simulink model "SimulationMobileManipulator"  (R2025b)
settings: Solver=FixedStepAuto  StartTime=0.0  StopTime=70  FixedStep=0.01  RelTol=1e-3  EnableMultiTasking=on
libraries: quarc_library x1
settings Model: ExtModeTrigDuration=10000  Creator=prata  LastModifiedBy=prata
settings SolverCC: AlgebraicLoopSolver=TrustRegion  PositivePriorityOrder=on
settings DataIOCC: ReturnWorkspaceOutputs=off
settings OptimizationCC: LifeSpan=inf
settings DebuggingCC: UnconnectedInputMsg=warning  UnconnectedOutputMsg=warning  UnconnectedLineMsg=warning  ArithmeticOperatorsInVariantConditions=warning
settings ModelReferenceCC: EnableRefExpFcnMdlSchedulingChecks=on
settings SFSimCC: SimUseLocalCustomCode=off  CustomCodeUndefinedFunction=UseInterfaceOnly
settings RTWCC: SystemTargetFile=quarc_win64.tlc  TemplateMakefile=quarc_default_tmf  RTWUseLocalCustomCode=off  GPUComputeCapability=3.5  Description=QUARC Win64 Target
settings CodeAppCC: StateflowObjectComments=on
settings STFCustomTargetCC: SystemTargetFile=quarc_win64.tlc  TargetPreCompLibLocation=C:\PROGRA~3\QUARC\lib\2016a\win64\release  TargetLangStandard=C99 (ISO)  DownloadToTarget=on  StopOnOverrun=off  Debug=off
settings GRTTargetCC: ExtMode=on  ExtModeMexFile=quarc_comm  TargetPreCompLibLocation=C:\PROGRA~3\QUARC\lib\2016a\win64\release  ParMdlRefBuildCompliant=off  CompOptLevelCompliant=off  CombineOutputUpdateFcns=off  MatFileLogging=off  CPPClassGenCompliant=off  GRTInterface=on  UseToolchainInfoCompliant=off
settings ConfigComp: CovMetricSettings=dswe

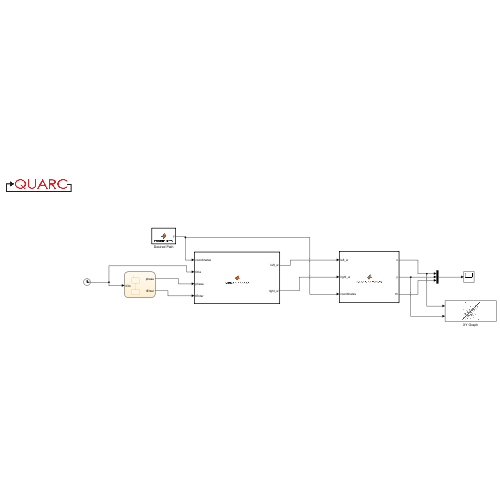
[thumbnail: Simulink's stored preview of the top-level diagram]
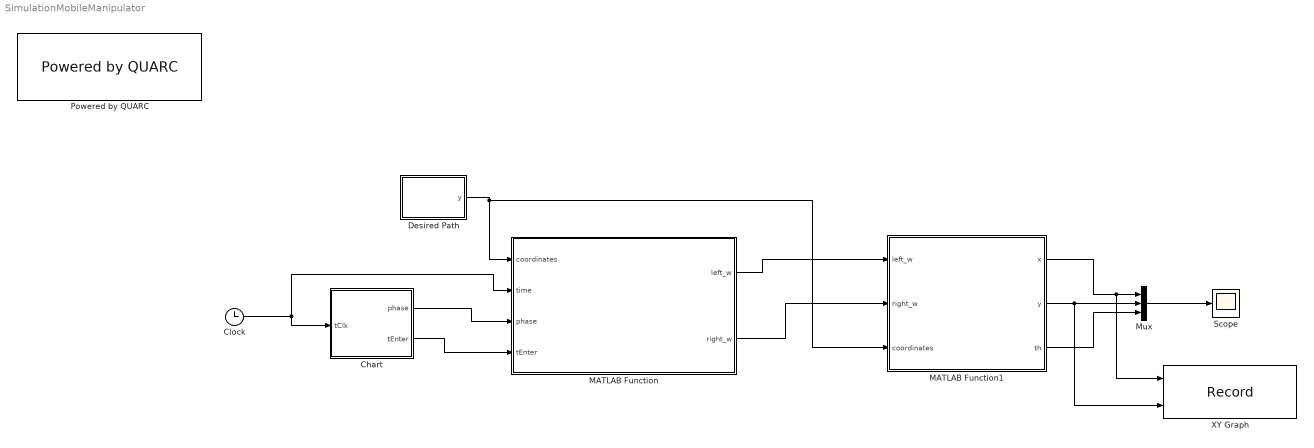
== system SimulationMobileManipulator ==
  Chart : Stateflow chart  TreatAsAtomicUnit=on
  Clock : Clock
  Desired Path : MATLAB Function  TreatAsAtomicUnit=on
  MATLAB Function : MATLAB Function  TreatAsAtomicUnit=on
  MATLAB Function1 : MATLAB Function  TreatAsAtomicUnit=on
  Mux : Mux  Inputs=3
  Powered by QUARC : quarc_library/Logos/Powered by QUARC
  Scope : Scope
      settings: ActiveDisplayYMinimum=-14.807697034096025  ActiveDisplayYMaximum=19.139251197660155
  XY Graph : Record  NumPorts=2.0  FileSettingsInternal="{\"entries\":[{\"content\":{\"excelSettings\":{\"content\":{},\"type\":\"Streamout.ExcelSettings\"},\"parquetSettings\":{\"content\":{},\"type\":\"Streamout.ParquetSettings\"}},\"type\":\"Streamout.FileSettingStorage\",\"uuid\":\"\"}],\"packageUris\":[\"http:\\/\\/schema.mathworks.com\\/mf0\\/streamout_blocks\\/R2020a\"],\"version\":\"1.0\"}"  FrameSettings=[0, 0]  Layout=[1 1]  SignalsInternal="{\"entries\":[{\"content\":{\"signals\":[{\"content\":{\"blockPath\":[],\"dimensions\":[1],\"domain\":\"\",\"lineColor\":\"#a2142f\",\"plots\":[ 1 ],\"port\":1,\"sid\":[\"\"],\"signalID\":1,\"signalName\":\"MATLAB Function1:1\"},\"type\":\"RecordBlkView.Signal\",\"uuid\":\"\"},{\"content\":{\"blockPath\":[],\"dimensions\":[1],\"domain\":\"\",\"lineColor\":\"#139fff\",\"plots\":[ 1 ],\"port\":2,\"sid\":[\"\"],\"signalID\":2,\"signalName\":\"MATLAB Function1:2\"},\"type\":\"RecordBlkView.Signal\",\"uuid\":\"\"}]},\"type\":\"RecordBlkView.InputSignals\",\"uuid\":\"\"}],\"packageUris\":[\"http:\\/\\/schema.mathworks.com\\/mf0\\/streamout_blocks\\/R2020a\"],\"version\":\"1.0\"}"  VisualizationBindings="{\"xyplotplugin\":{\"info\":[{\"series\":[{\"bindingParametersList\":[{\"parameter\":\"X-Axis\",\"signalID\":1,\"signalName\":\"MATLAB Function1:1\"},{\"parameter\":\"Y-Axis\",\"signalID\":2,\"signalName\":\"MATLAB Function1:2\"}],\"seriesID\":0}],\"subplotID\":1}]}}"  CompatibilityTag=XY
  wires:
  Desired Path/1(y) -> MATLAB Function1/3(coordinates), MATLAB Function/1(coordinates)
  Chart/1(phase) -> MATLAB Function/3(phase)
  Chart/2(tEnter) -> MATLAB Function/4(tEnter)
  Clock/1 -> MATLAB Function/2(time), Chart/1(tClk)
  MATLAB Function/1(left_w) -> MATLAB Function1/1(left_w)
  MATLAB Function/2(right_w) -> MATLAB Function1/2(right_w)
  MATLAB Function1/2(y) -> XY Graph/2, Mux/2
  MATLAB Function1/1(x) -> XY Graph/1, Mux/1
  MATLAB Function1/3(th) -> Mux/3
  Mux/1 -> Scope/1

== matlab function SimulationMobileManipulator/Desired Path ==
  data: y output
function y = coordinates()
a = 1.0;                      % half-width of the loop (m)
N = 200;                      % number of waypoints
t = linspace(0, 2*pi, N)';
d = 1 + sin(t).^2;
y = [a*cos(t)./d, a*sin(t).*cos(t)./d];   % [x y], N-by-2
end

== matlab function SimulationMobileManipulator/MATLAB Function ==
  data: left_w output; coordinates input; time input; phase input; tEnter input; right_w output
function [left_w, right_w] = MissionPlanner(coordinates, time, phase, tEnter)
% left_w / right_w = [dirn, speed]   (dirn = +1 forward, -1 reverse)
b     = 0.235;     % wheel track width (m)
v_ref = 0.2;       % forward speed (m/s)

left_w  = [1, 0];
right_w = [1, 0];

if phase ~= 1
    return;                              % Settle: hold still
end

tp  = max(time - tEnter, 0);
N   = size(coordinates, 1);

seg = coordinates(2:end,:) - coordinates(1:end-1,:);
len = sqrt(sum(seg.^2, 2));
cum = [0; cumsum(len)];

k = sum(cum <= v_ref * tp);

if k > N-2
    return;                              % end of path: stop
end

h1 = atan2(seg(k,2),   seg(k,1));
h2 = atan2(seg(k+1,2), seg(k+1,1));
dh = atan2(sin(h2-h1), cos(h2-h1));

omega = dh / (len(k) / v_ref);

vL = v_ref - omega*b/2;
vR = v_ref + omega*b/2;

left_w  = [2*(vL >= 0) - 1, abs(vL)];
right_w = [2*(vR >= 0) - 1, abs(vR)];
end

== stateflow chart SimulationMobileManipulator/Chart ==
  state Settle
    entry:
    phase = 0;
    tEnter = tClk;
  state Trace
    entry:
    phase = 1;
    tEnter = tClk;
  (default) -> Settle
  Settle -> Trace : [tClk - tEnter >= 26.1]
  data: tClk input; phase output; tEnter output; ChartMode local Enum: ChartModeType

== matlab function SimulationMobileManipulator/MATLAB Function1 ==
  data: x output; left_w input; y output; right_w input; coordinates input; th output
function [x, y, th] = BaseKinematics(left_w, right_w, coordinates)
persistent X Y TH
dt = 0.01;  b = 0.235;                       % must match solver step and planner
if isempty(X)
    X = coordinates(1,1);  Y = coordinates(1,2);
    TH = atan2(coordinates(2,2)-coordinates(1,2), coordinates(2,1)-coordinates(1,1));
end
vL = left_w(1)*left_w(2);
vR = right_w(1)*right_w(2);
v  = (vL + vR)/2;
om = (vR - vL)/b;
X  = X  + v*cos(TH)*dt;
Y  = Y  + v*sin(TH)*dt;
TH = TH + om*dt;
x = X;  y = Y;  th = TH;
end
